simulink model "Router_communication"  (R2025a)
settings: Solver=VariableStepAuto  StartTime=0.0  StopTime=30  RelTol=1e-3
InitFcn:
  | %% Simulation parameters and waypoint trajectory
  | % Initial drone positions.
  | init_0=[0;0;0];
  | d_s=4;
  | init_1=init_0+d_s*[-1.1;0.1;0];
  | init_2=init_0+d_s*[0.3;-1.5;0];
  | init_3=init_0+d_s*[0.2;1.8;0];
  | init_4=init_0+d_s*[1.6;0.4;0];
  | 
  | Threshold = 1000*ones(45,1);
  | for i=1:9:37
  |     Threshold(i:i+2)=10;
  | end
  | gain_2=1;
  | 
  | % Router queues and background traffic.
  | router_buffer=5;
  | router_bandwith=20;
  | router_init_queue=3;
  | traffic_mean=20;
  | traffic_variance=1;
  | 
  | 
  | % Desired formation offsets.
  | init_f_0=[0;0;0];
  | d_f=1;
  | init_f_1=init_0+d_f*[-1;0;0];
  | init_f_2=init_0+d_f*[0;-1;0];
  | init_f_3=init_0+d_f*[0;1;0];
  | init_f_4=init_0+d_f*[1;0;0];
  | 
  | % Quadrotor mass and inertia.
  | mass = 1.2;
  | Ib   = diag([1.2416 1.2416 2*1.2416]);
  | 
  | % Time grid and waypoint trajectory.
  | Ts        = 0.001;
  | ttot      = 20;
  | tdead     = 10;
  | totalTime = ttot + tdead;
  | Nsamples  = 3000;
  | t_sample  = linspace(0, totalTime, Nsamples);
  | t=t_sample;
  | waypoints = [ ...
  |              0  0 -2 0;
  |              3  4 -5 0;
  |              2  1 -8 0;
  |              0 0 -10 0];
  | 
  | M    = size(waypoints,1);
  | t_wp = linspace(0, ttot, M);
  | 
  | p_d      = zeros(4, Nsamples);
  | dot_p_d  = zeros(4, Nsamples);
  | ddot_p_d = zeros(4, Nsamples);
  | 
  | idx_traj = t_sample <= ttot;
  | t_active = t_sample(idx_traj);
  | 
  | % Build position and yaw splines with zero endpoint velocities.
  | for dim = 1:4
  |     pp  = spline(t_wp, [0, waypoints(:,dim)&apos;, 0]);
  |     pp1 = fnder(pp,1);
  |     pp2 = fnder(pp,2);
  | 
  |     p_d(dim,    idx_traj) = ppval(pp,  t_active);
  |     dot_p_d(dim,idx_traj) = ppval(pp1, t_active);
  |     ddot_p_d(dim,idx_traj)= ppval(pp2, t_active);
  | end
  | 
  | % Hold the final waypoint after the maneuver.
  | last_wp_idx = M;
  | p_d(:, ~idx_traj)      = repmat(waypoints(last_wp_idx,:)&apos;, 1, sum(~idx_traj));
  | dot_p_d(:, ~idx_traj)  = 0;
  | ddot_p_d(:, ~idx_traj) = 0;
  | 
  | % Reference signals used by the Simulink blocks.
  | csi_d      = p_d(1:3,:);
  | psi_d      = p_d(4,:);
  | 
  | dot_csi_d  = dot_p_d(1:3,:);
  | ddot_csi_d = ddot_p_d(1:3,:);
  | dot_psi_d  = dot_p_d(4,:);
  | ddot_psi_d = ddot_p_d(4,:);
  | 
  | pos_0     = waypoints(1,1:3);
  | lin_vel_0 = [0 0 0];
  | w_bb_0    = [0 0 0];
undefined symbols (not defined in the file): A_diacenza, K
libraries: robotcorelib x5, dspsigops x1, uavutilslib x1
(part 1 of 3)
settings Model: Creator=fabioruggiero  LastModifiedBy=Giammo
settings ModelReferenceCC: EnableRefExpFcnMdlSchedulingChecks=on
settings RTWCC: GPUComputeCapability=3.5

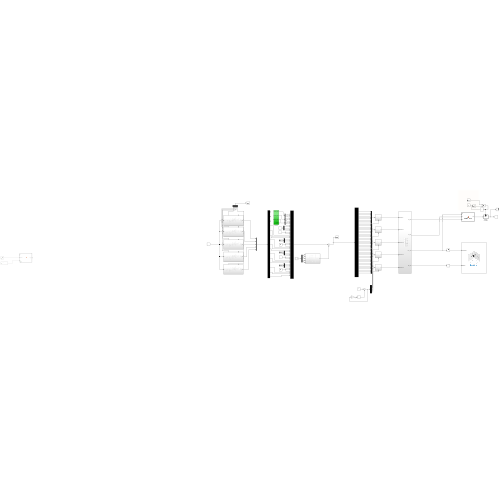
[thumbnail: Simulink's stored preview of the top-level diagram]
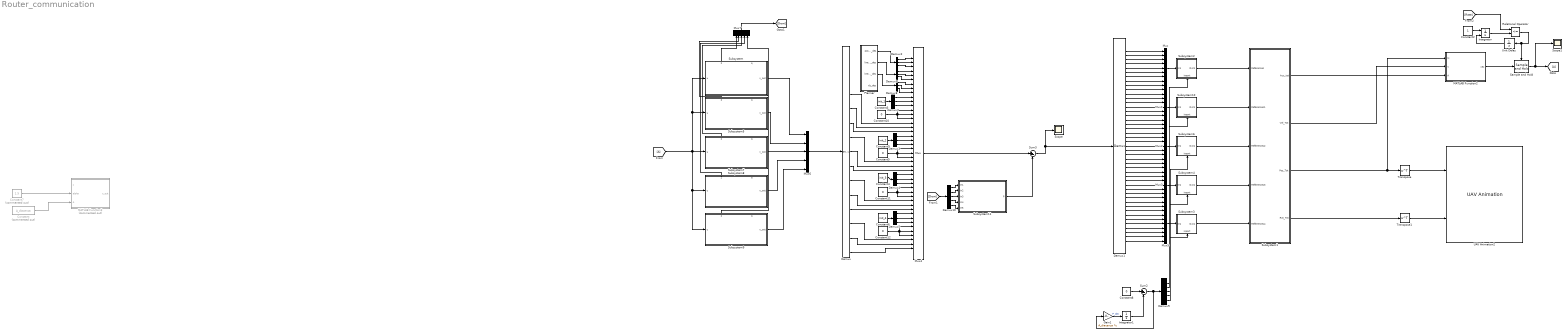
== system Router_communication ==
  Constant : Constant  Commented=on  Value=A_diacenza
  Constant{5,8,10..12} (5 alike) : Constant  Value=0
  Constant2 : Constant
  Constant3 : Constant  Value=init_1
  Constant4 : Constant  Value=init_3
  Constant6 : Constant  Value=init_4
  Constant7 : Constant  Commented=on  Value=1.5
  Constant9 : Constant  Value=init_2
  Demux : Demux  Outputs=15
  Demux1 : Demux  Outputs=45
  Demux10 : Demux  Outputs=5
  Demux{2..8} (7 alike) : Demux  Outputs=3
  Demux9 : Demux  Outputs=5
  From : From
  Gain1 : Gain  Gain=A_diacenza  Multiplication=Matrix(K*u)
  Goto : Goto
  Integrator : Integrator  ExternalReset=rising
  Integrator1 : Integrator
  MATLAB Function2 : MATLAB Function  TreatAsAtomicUnit=on
  MATLAB Function3 : MATLAB Function  Commented=on  TreatAsAtomicUnit=on
  Mux{,1..3,5} (5 alike) : Mux  Inputs=9
  Mux4 : Mux  Inputs=45
  Mux6 : Mux  Inputs=5
  Mux7 : Mux  Inputs=5
  Planner : Subsystem
  Relational Operator : RelationalOperator  Operator=<=  OutDataTypeStr=boolean  RndMeth=Simplest  InputSameDT=off
  Sample and Hold : dspsigops/Sample and Hold  trig=Rising edge  initCond=0  latchinput=off
  Scope : Scope
      settings: ActiveDisplayYMinimum=-34.636381337350009  ActiveDisplayYMaximum=35.165535436651609  DataLoggingVariableName=ScopeData6
  Scope1 : Scope
      settings: ActiveDisplayYMinimum=-11.627869915109368  ActiveDisplayYMaximum=11.845520962750264  DataLoggingVariableName=ScopeData33
  Subsystem : Subsystem
      settings: PortSchema="{\"entries\":[{\"content\":{\"sides\":[{\"content\":{\"connectorIds\":[\"In1\"]},\"type\":\"ConnectorPlacement.EquallySpacedRectSide\",\"uuid\":\"aabcef1b-4fc2-4bd0-92ff-98af5bae71df\"},{\"content\":{\"connectorIds\":[\"Out1\"],\"side\":\"RIGHT\"},\"type\":\"ConnectorPlacement.EquallySpacedRectSide\",\"uuid\":\"7f481425-bc3c-4684-b5b9-3c38277c27e3\"},{\"content\":{\"connectorIds\":[\"Out2\",\"Out3\"],\"side\":\"TOP\"},\"type\":\"ConnectorPlacement.EquallySpacedRectSide\",\"uuid\":\"89424cd8-205b-4e4e-84ff-a3a586731ce6\"}]},\"type\":\"ConnectorPlacement.EquallySpacedConnector\",\"uuid\":\"cde5d1e6-587e-462f-b172-cbaeaf24433c\"}],\"packageUris\":[\"http://schema.mathworks.com/mf0/Connector/R2020b\"],\"version\":\"1.0\"}"
  Subsystem1 : Subsystem
  Subsystem10 : Subsystem
      settings: PortSchema="{\"entries\":[{\"content\":{\"sides\":[{\"content\":{\"connectorIds\":[\"In1\"]},\"type\":\"ConnectorPlacement.EquallySpacedRectSide\",\"uuid\":\"6e5d8b99-8054-458f-abbe-7e3d6126420c\"},{\"content\":{\"connectorIds\":[\"Out1\"],\"side\":\"RIGHT\"},\"type\":\"ConnectorPlacement.EquallySpacedRectSide\",\"uuid\":\"d8af8c34-1227-4a19-bfdc-b42d943ed13c\"},{\"content\":{\"side\":\"TOP\"},\"type\":\"ConnectorPlacement.EquallySpacedRectSide\",\"uuid\":\"9c10b933-2873-4349-b535-f2af5c16ec70\"},{\"content\":{\"connectorIds\":[\"In2\"],\"side\":\"BOTTOM\"},\"type\":\"ConnectorPlacement.EquallySpacedRectSide\",\"uuid\":\"05be8d01-ed26-4f96-bcb1-0e501cb43bcc\"}]},\"type\":\"ConnectorPlacement.EquallySpacedConnector\",\"uuid\":\"f87e25de-488b-44c6-b2e5-9d22d609821c\"}],\"packageUris\":[\"http://schema.mathworks.com/mf0/Connector/R2020b\"],\"version\":\"1.0\"}"
  Subsystem11 : Subsystem
  Subsystem2 : Subsystem
      settings: PortSchema="{\"entries\":[{\"content\":{\"sides\":[{\"content\":{\"connectorIds\":[\"In1\"]},\"type\":\"ConnectorPlacement.EquallySpacedRectSide\",\"uuid\":\"6e5d8b99-8054-458f-abbe-7e3d6126420c\"},{\"content\":{\"connectorIds\":[\"Out1\"],\"side\":\"RIGHT\"},\"type\":\"ConnectorPlacement.EquallySpacedRectSide\",\"uuid\":\"d8af8c34-1227-4a19-bfdc-b42d943ed13c\"},{\"content\":{\"side\":\"TOP\"},\"type\":\"ConnectorPlacement.EquallySpacedRectSide\",\"uuid\":\"9c10b933-2873-4349-b535-f2af5c16ec70\"},{\"content\":{\"connectorIds\":[\"In2\"],\"side\":\"BOTTOM\"},\"type\":\"ConnectorPlacement.EquallySpacedRectSide\",\"uuid\":\"05be8d01-ed26-4f96-bcb1-0e501cb43bcc\"}]},\"type\":\"ConnectorPlacement.EquallySpacedConnector\",\"uuid\":\"f87e25de-488b-44c6-b2e5-9d22d609821c\"}],\"packageUris\":[\"http://schema.mathworks.com/mf0/Connector/R2020b\"],\"version\":\"1.0\"}"
  Subsystem3 : Subsystem
      settings: PortSchema="{\"entries\":[{\"content\":{\"sides\":[{\"content\":{\"connectorIds\":[\"In1\"]},\"type\":\"ConnectorPlacement.EquallySpacedRectSide\",\"uuid\":\"6e5d8b99-8054-458f-abbe-7e3d6126420c\"},{\"content\":{\"connectorIds\":[\"Out1\"],\"side\":\"RIGHT\"},\"type\":\"ConnectorPlacement.EquallySpacedRectSide\",\"uuid\":\"d8af8c34-1227-4a19-bfdc-b42d943ed13c\"},{\"content\":{\"side\":\"TOP\"},\"type\":\"ConnectorPlacement.EquallySpacedRectSide\",\"uuid\":\"9c10b933-2873-4349-b535-f2af5c16ec70\"},{\"content\":{\"connectorIds\":[\"In2\"],\"side\":\"BOTTOM\"},\"type\":\"ConnectorPlacement.EquallySpacedRectSide\",\"uuid\":\"05be8d01-ed26-4f96-bcb1-0e501cb43bcc\"}]},\"type\":\"ConnectorPlacement.EquallySpacedConnector\",\"uuid\":\"f87e25de-488b-44c6-b2e5-9d22d609821c\"}],\"packageUris\":[\"http://schema.mathworks.com/mf0/Connector/R2020b\"],\"version\":\"1.0\"}"
  Subsystem4 : Subsystem
      settings: PortSchema="{\"entries\":[{\"content\":{\"sides\":[{\"content\":{\"connectorIds\":[\"In1\"]},\"type\":\"ConnectorPlacement.EquallySpacedRectSide\",\"uuid\":\"6e5d8b99-8054-458f-abbe-7e3d6126420c\"},{\"content\":{\"connectorIds\":[\"Out1\"],\"side\":\"RIGHT\"},\"type\":\"ConnectorPlacement.EquallySpacedRectSide\",\"uuid\":\"d8af8c34-1227-4a19-bfdc-b42d943ed13c\"},{\"content\":{\"side\":\"TOP\"},\"type\":\"ConnectorPlacement.EquallySpacedRectSide\",\"uuid\":\"9c10b933-2873-4349-b535-f2af5c16ec70\"},{\"content\":{\"connectorIds\":[\"In2\"],\"side\":\"BOTTOM\"},\"type\":\"ConnectorPlacement.EquallySpacedRectSide\",\"uuid\":\"05be8d01-ed26-4f96-bcb1-0e501cb43bcc\"}]},\"type\":\"ConnectorPlacement.EquallySpacedConnector\",\"uuid\":\"f87e25de-488b-44c6-b2e5-9d22d609821c\"}],\"packageUris\":[\"http://schema.mathworks.com/mf0/Connector/R2020b\"],\"version\":\"1.0\"}"
  Subsystem5 : Subsystem
      settings: PortSchema="{\"entries\":[{\"content\":{\"sides\":[{\"content\":{\"connectorIds\":[\"In1\"]},\"type\":\"ConnectorPlacement.EquallySpacedRectSide\",\"uuid\":\"aabcef1b-4fc2-4bd0-92ff-98af5bae71df\"},{\"content\":{\"connectorIds\":[\"Out1\"],\"side\":\"RIGHT\"},\"type\":\"ConnectorPlacement.EquallySpacedRectSide\",\"uuid\":\"7f481425-bc3c-4684-b5b9-3c38277c27e3\"},{\"content\":{\"connectorIds\":[\"Out2\",\"Out3\"],\"side\":\"TOP\"},\"type\":\"ConnectorPlacement.EquallySpacedRectSide\",\"uuid\":\"89424cd8-205b-4e4e-84ff-a3a586731ce6\"}]},\"type\":\"ConnectorPlacement.EquallySpacedConnector\",\"uuid\":\"cde5d1e6-587e-462f-b172-cbaeaf24433c\"}],\"packageUris\":[\"http://schema.mathworks.com/mf0/Connector/R2020b\"],\"version\":\"1.0\"}"
  Subsystem6 : Subsystem
      settings: PortSchema="{\"entries\":[{\"content\":{\"sides\":[{\"content\":{\"connectorIds\":[\"In1\"]},\"type\":\"ConnectorPlacement.EquallySpacedRectSide\",\"uuid\":\"6e5d8b99-8054-458f-abbe-7e3d6126420c\"},{\"content\":{\"connectorIds\":[\"Out1\"],\"side\":\"RIGHT\"},\"type\":\"ConnectorPlacement.EquallySpacedRectSide\",\"uuid\":\"d8af8c34-1227-4a19-bfdc-b42d943ed13c\"},{\"content\":{\"side\":\"TOP\"},\"type\":\"ConnectorPlacement.EquallySpacedRectSide\",\"uuid\":\"9c10b933-2873-4349-b535-f2af5c16ec70\"},{\"content\":{\"connectorIds\":[\"In2\"],\"side\":\"BOTTOM\"},\"type\":\"ConnectorPlacement.EquallySpacedRectSide\",\"uuid\":\"05be8d01-ed26-4f96-bcb1-0e501cb43bcc\"}]},\"type\":\"ConnectorPlacement.EquallySpacedConnector\",\"uuid\":\"f87e25de-488b-44c6-b2e5-9d22d609821c\"}],\"packageUris\":[\"http://schema.mathworks.com/mf0/Connector/R2020b\"],\"version\":\"1.0\"}"
  Subsystem7 : Subsystem
      settings: PortSchema="{\"entries\":[{\"content\":{\"sides\":[{\"content\":{\"connectorIds\":[\"In1\"]},\"type\":\"ConnectorPlacement.EquallySpacedRectSide\",\"uuid\":\"aabcef1b-4fc2-4bd0-92ff-98af5bae71df\"},{\"content\":{\"connectorIds\":[\"Out1\"],\"side\":\"RIGHT\"},\"type\":\"ConnectorPlacement.EquallySpacedRectSide\",\"uuid\":\"7f481425-bc3c-4684-b5b9-3c38277c27e3\"},{\"content\":{\"connectorIds\":[\"Out2\",\"Out3\"],\"side\":\"TOP\"},\"type\":\"ConnectorPlacement.EquallySpacedRectSide\",\"uuid\":\"89424cd8-205b-4e4e-84ff-a3a586731ce6\"}]},\"type\":\"ConnectorPlacement.EquallySpacedConnector\",\"uuid\":\"cde5d1e6-587e-462f-b172-cbaeaf24433c\"}],\"packageUris\":[\"http://schema.mathworks.com/mf0/Connector/R2020b\"],\"version\":\"1.0\"}"
  Subsystem8 : Subsystem
      settings: PortSchema="{\"entries\":[{\"content\":{\"sides\":[{\"content\":{\"connectorIds\":[\"In1\"]},\"type\":\"ConnectorPlacement.EquallySpacedRectSide\",\"uuid\":\"aabcef1b-4fc2-4bd0-92ff-98af5bae71df\"},{\"content\":{\"connectorIds\":[\"Out1\"],\"side\":\"RIGHT\"},\"type\":\"ConnectorPlacement.EquallySpacedRectSide\",\"uuid\":\"7f481425-bc3c-4684-b5b9-3c38277c27e3\"},{\"content\":{\"connectorIds\":[\"Out2\",\"Out3\"],\"side\":\"TOP\"},\"type\":\"ConnectorPlacement.EquallySpacedRectSide\",\"uuid\":\"89424cd8-205b-4e4e-84ff-a3a586731ce6\"}]},\"type\":\"ConnectorPlacement.EquallySpacedConnector\",\"uuid\":\"cde5d1e6-587e-462f-b172-cbaeaf24433c\"}],\"packageUris\":[\"http://schema.mathworks.com/mf0/Connector/R2020b\"],\"version\":\"1.0\"}"
  Subsystem9 : Subsystem
      settings: PortSchema="{\"entries\":[{\"content\":{\"sides\":[{\"content\":{\"connectorIds\":[\"In1\"]},\"type\":\"ConnectorPlacement.EquallySpacedRectSide\",\"uuid\":\"c75a44b6-9c90-4115-8324-491a5ed9c89c\"},{\"content\":{\"connectorIds\":[\"Out1\"],\"side\":\"RIGHT\"},\"type\":\"ConnectorPlacement.EquallySpacedRectSide\",\"uuid\":\"690e00bc-d919-4544-9758-30244acb19c7\"},{\"content\":{\"connectorIds\":[\"Out2\",\"Out3\"],\"side\":\"TOP\"},\"type\":\"ConnectorPlacement.EquallySpacedRectSide\",\"uuid\":\"5c005ee2-f6aa-4388-a92a-4c7221a2c358\"}]},\"type\":\"ConnectorPlacement.EquallySpacedConnector\",\"uuid\":\"c7f8f7aa-2ed0-42e7-91ea-44ddde2a21e1\"}],\"packageUris\":[\"http://schema.mathworks.com/mf0/Connector/R2020b\"],\"version\":\"1.0\"}"
  Sum2 : Sum  Inputs=|+-
  Sum3 : Sum  Inputs=|+-
  Transpose : Math  Operator=transpose
  Transpose1 : Math  Operator=transpose
  UAV Animation2 : uavutilslib/UAV Animation  NumUAV=5  DynamicUAVConfig=off  UAVType=Multirotor  UAVSize=1  UAVColor=[1 0 0]  UAVTrajectoryAlpha=1  InertialZDirection=Down  RotationFormat=Quaternion  DrawMarkers=off  SampleTime=0.01
  Unit Delay : UnitDelay  SampleTime=Ts  HasFrameUpgradeWarning=on
  wires:
  Demux9/5 -> Subsystem3/2(Inport)
  Transpose1/1 -> UAV Animation2/2
  Transpose/1 -> UAV Animation2/1
  Sum2/1 -> Demux9/1, Gain1/1
  Gain1/1 -> Integrator1/1  "P_dot"
  Integrator1/1 -> Sum2/2
  Mux3/1 -> Subsystem4/1(In1)
  Mux/1 -> Subsystem2/1(In1)
  Subsystem2/1(Out1) -> Subsystem1/1(References)
  Demux9/2 -> Subsystem10/2(Inport)
  Subsystem3/1(Out1) -> Subsystem1/5(References4)
  Mux5/1 -> Subsystem3/1(In1)
  Subsystem6/1(Out1) -> Subsystem1/3(References2)
  Mux2/1 -> Subsystem6/1(In1)
  Demux1/1 -> Mux/1
  Demux1/15 -> Mux1/6
  Demux9/1 -> Subsystem2/2(Inport)
  Demux1/23 -> Mux2/5
  Demux1/12 -> Mux1/3
  Demux1/4 -> Mux/4
  Demux1/31 -> Mux3/4
  Demux1/41 -> Mux5/5
  Demux1/19 -> Mux2/1
  Demux1/26 -> Mux2/8
  Demux1/29 -> Mux3/2
  Demux1/34 -> Mux3/7
  Demux1/39 -> Mux5/3
  Demux1/20 -> Mux2/2
  Demux1/38 -> Mux5/2
  Demux1/43 -> Mux5/7
  Demux1/42 -> Mux5/6
  Demux1/30 -> Mux3/3
  Demux1/36 -> Mux3/9
  Demux1/27 -> Mux2/9
  Demux9/4 -> Subsystem4/2(Inport)
  Demux1/22 -> Mux2/4
  Demux1/32 -> Mux3/5
  Demux1/14 -> Mux1/5
  Demux1/13 -> Mux1/4
  Demux1/21 -> Mux2/3
  Demux1/33 -> Mux3/6
  Subsystem1/4(Rot_Tot) -> Transpose1/1
  Demux1/9 -> Mux/9
  Mux1/1 -> Subsystem10/1(In1)
  Demux1/40 -> Mux5/4
  Demux1/3 -> Mux/3
  Demux1/6 -> Mux/6
  Demux1/25 -> Mux2/7
  Demux1/8 -> Mux/8
  Demux1/28 -> Mux3/1
  Demux1/10 -> Mux1/1
  Demux1/7 -> Mux/7
  Demux1/37 -> Mux5/1
  Demux1/11 -> Mux1/2
  Demux1/45 -> Mux5/9
  Demux1/17 -> Mux1/8
  Demux1/35 -> Mux3/8
  Demux1/5 -> Mux/5
  Demux1/44 -> Mux5/8
  Constant11/1 -> Mux4/31, Mux4/33, Mux4/32
  Planner/3(linear_acceleration_des) -> Demux8/1
  Demux1/18 -> Mux1/9
  Demux/9 -> Mux4/27
  Demux1/16 -> Mux1/7
  Demux1/2 -> Mux/2
  Constant7/1 -> MATLAB Function3/2(alpha)
  Constant12/1 -> Mux4/40, Mux4/41, Mux4/42
  Constant10/1 -> Mux4/13, Mux4/15, Mux4/14
  Demux4/3 -> Mux4/30
  Mux4/1 -> Sum3/1
  Demux3/2 -> Mux4/20
  Demux2/2 -> Mux4/2
  Constant3/1 -> Demux7/1
  Demux5/2 -> Mux4/38
  Demux8/2 -> Mux4/8
  Constant8/1 -> Sum2/1
  Demux2/1 -> Mux4/1
  Demux7/2 -> Mux4/11
  Demux8/1 -> Mux4/7
  Demux2/3 -> Mux4/3
  Constant5/1 -> Mux4/22, Mux4/24, Mux4/23
  Demux/6 -> Mux4/18
  Demux3/3 -> Mux4/21
  Demux6/1 -> Mux4/4
  Demux/5 -> Mux4/17
  Demux8/3 -> Mux4/9
  Demux/12 -> Mux4/36
  Constant4/1 -> Demux4/1
  Demux6/2 -> Mux4/5
  Demux/7 -> Mux4/25
  Demux/14 -> Mux4/44
  Constant6/1 -> Demux5/1
  Constant9/1 -> Demux3/1
  Demux5/3 -> Mux4/39
  Demux/8 -> Mux4/26
  Demux7/1 -> Mux4/10
  Demux7/3 -> Mux4/12
  Planner/2(linear_velocity_des) -> Demux6/1
  Constant/1 -> MATLAB Function3/3(A)
  Sum3/1 -> Demux1/1, Scope/1
  Subsystem4/1(Out1) -> Subsystem1/4(References3)
  Demux3/1 -> Mux4/19
  Demux4/1 -> Mux4/28
  Demux4/2 -> Mux4/29
  Demux/10 -> Mux4/34
  Demux6/3 -> Mux4/6
  Demux/4 -> Mux4/16
  Planner/1(position_des) -> Demux2/1
  Demux5/1 -> Mux4/37
  Demux/11 -> Mux4/35
  Demux/15 -> Mux4/45
  Demux9/3 -> Subsystem6/2(Inport)
  Demux1/24 -> Mux2/6
  Subsystem10/1(Out1) -> Subsystem1/2(References1)
  Demux/13 -> Mux4/43
  Subsystem1/3(Pos_Tot) -> MATLAB Function2/1(M), Transpose/1
  Subsystem1/2(Vel_Tot) -> MATLAB Function2/2(V)
  Subsystem1/1(Acc_tot) -> MATLAB Function2/3(A)
  Mux6/1 -> Demux/1
  Subsystem/1(v_out) -> Mux6/1
  Subsystem5/1(v_out) -> Mux6/2
  Subsystem7/1(v_out) -> Mux6/3
  Subsystem8/1(v_out) -> Mux6/4
  Subsystem9/1(v_out) -> Mux6/5
  Subsystem11/1(P) -> Sum3/2
  Subsystem/2(" ") -> Mux7/1
  Demux10/1 -> Subsystem11/1(In1)
  Demux10/2 -> Subsystem11/2(In2)
  Demux10/3 -> Subsystem11/3(In3)
  Demux10/4 -> Subsystem11/4(In4)
  Demux10/5 -> Subsystem11/5(In5)
  Subsystem5/2(" ") -> Mux7/2
  Subsystem7/2(" ") -> Mux7/3
  Subsystem8/2(" ") -> Mux7/4
  Subsystem9/2(" ") -> Mux7/5
  Mux7/1 -> [Droni]
  [Droni] -> Demux10/1
  From/1 -> Subsystem7/1(u), Subsystem/1(u), Subsystem5/1(u), Subsystem8/1(u), Subsystem9/1(u)
  Constant2/1 -> Integrator/1
  Integrator/1 -> Relational Operator/2
  Relational Operator/1 -> Sample and Hold/Trigger, Unit Delay/1
  MATLAB Function2/1(vec) -> Sample and Hold/1
  Unit Delay/1 -> Integrator/2
  Sample and Hold/1 -> Scope1/1, Goto/1
  [Rate] -> Relational Operator/1

== system Router_communication/Planner ==
  Constant : Constant  Value=0
  Mux{1..4} (4 alike) : Mux  Inputs=3
  Trigonometric Function : Trigonometry
  Trigonometric Function1 : Trigonometry  Operator=cos
  ddot_x_d : FromWorkspace  VariableName=[t' ddot_csi_d(1,:)']  SampleTime=Ts
  ddot_y_d : FromWorkspace  VariableName=[t' ddot_csi_d(2,:)']  SampleTime=Ts
  ddot_z_d : FromWorkspace  VariableName=[t' ddot_csi_d(3,:)']  SampleTime=Ts
  dot_x_d1 : FromWorkspace  VariableName=[t' dot_csi_d(1,:)']  SampleTime=Ts
  dot_y_d1 : FromWorkspace  VariableName=[t' dot_csi_d(2,:)']  SampleTime=Ts
  dot_z_d1 : FromWorkspace  VariableName=[t' dot_csi_d(3,:)']  SampleTime=Ts
  psi_d1 : FromWorkspace  VariableName=[t' psi_d']  SampleTime=Ts
  x_d : FromWorkspace  VariableName=[t' csi_d(1,:)']  SampleTime=Ts
  y_d : FromWorkspace  VariableName=[t' csi_d(2,:)']  SampleTime=Ts
  z_d : FromWorkspace  VariableName=[t' csi_d(3,:)']  SampleTime=Ts
  position_des : Outport
  linear_velocity_des : Outport  Port=2
  linear_acceleration_des : Outport  Port=3
  xb_des : Outport  Port=4
  wires:
  y_d/1 -> Mux1/2
  z_d/1 -> Mux1/3
  x_d/1 -> Mux1/1
  ddot_y_d/1 -> Mux2/2
  ddot_z_d/1 -> Mux2/3
  ddot_x_d/1 -> Mux2/1
  Mux2/1 -> linear_acceleration_des/1
  Mux1/1 -> position_des/1
  dot_y_d1/1 -> Mux3/2
  dot_z_d1/1 -> Mux3/3
  dot_x_d1/1 -> Mux3/1
  Mux3/1 -> linear_velocity_des/1
  Mux4/1 -> xb_des/1
  Trigonometric Function/1 -> Mux4/2
  psi_d1/1 -> Trigonometric Function/1, Trigonometric Function1/1
  Trigonometric Function1/1 -> Mux4/1
  Constant/1 -> Mux4/3

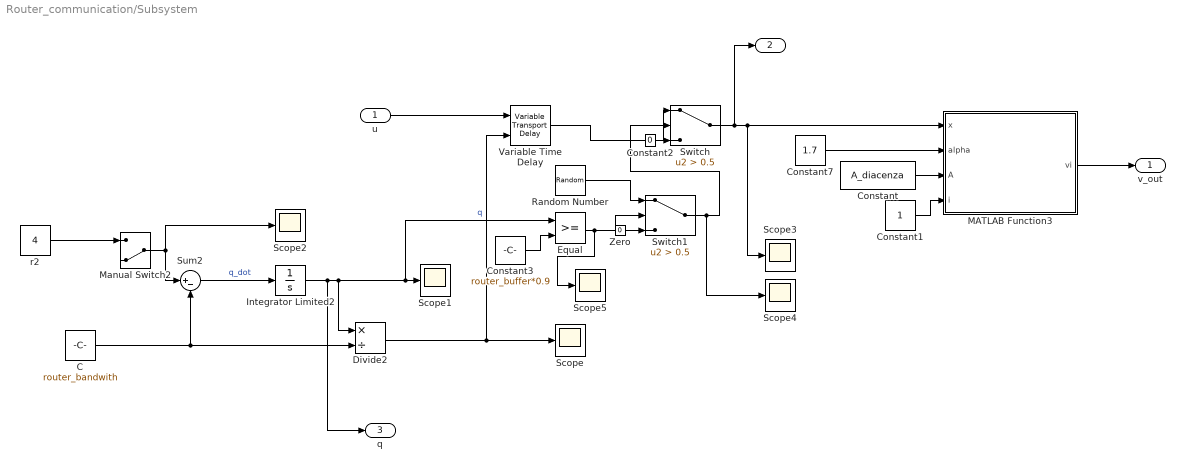
== system Router_communication/Subsystem ==
  u : Inport
  C : Constant  Value=router_bandwith
  Constant : Constant  Value=A_diacenza
  Constant1 : Constant
  Constant2 : Constant  Value=0
  Constant3 : Constant  Value=router_buffer*0.9
  Constant7 : Constant  Value=1.7
  Divide2 : Product  Inputs=*/
  Equal : RelationalOperator  OutDataTypeStr=boolean  RndMeth=Simplest  InputSameDT=off
  Integrator Limited2 : Integrator  InitialCondition=router_init_queue  LimitOutput=on  UpperSaturationLimit=router_buffer  LowerSaturationLimit=0
  MATLAB Function3 : MATLAB Function  TreatAsAtomicUnit=on
  Manual Switch2 : ManualSwitch  CurrentSetting=0
  Random Number : RandomNumber  Mean=0.5  SampleTime=0.1
  Scope{,1..5} (6 alike) : Scope
      Scope settings: ActiveDisplayYMinimum=0.1590289216839415  ActiveDisplayYMaximum=0.16563506037620399  DataLoggingVariableName=ScopeData7
      Scope1 settings: ActiveDisplayYMinimum=-1  ActiveDisplayYMaximum=1  DataLoggingVariableName=ScopeData8
      Scope2 settings: ActiveDisplayYMinimum=-4.9431007592698686  ActiveDisplayYMaximum=10.428917159954647  DataLoggingVariableName=ScopeData13
      Scope3 settings: ActiveDisplayYMinimum=-158.42328908870167  ActiveDisplayYMaximum=167.3995112416481  DataLoggingVariableName=ScopeData14
      Scope4 settings: ActiveDisplayYMinimum=-1  ActiveDisplayYMaximum=1  DataLoggingVariableName=ScopeData17
      Scope5 settings: ActiveDisplayYMinimum=-1  ActiveDisplayYMaximum=1  DataLoggingVariableName=ScopeData32
  Sum2 : Sum  Inputs=|+-
  Switch : Switch  Criteria=u2 > Threshold  Threshold=0.5  SaturateOnIntegerOverflow=off  InputSameDT=off
  Switch1 : Switch  Criteria=u2 > Threshold  Threshold=0.5  SaturateOnIntegerOverflow=off  InputSameDT=off
  Variable Time Delay : VariableTransportDelay  MaximumDelay=1000  InitialOutput=[init_0;zeros(6,1);init_1;zeros(6,1);init_2;zeros(6,1);init_3;zeros(6,1);init_4;zeros(6,1);]  MaximumPoints=1e4  ZeroDelay=on
  Zero : Constant  Value=0  OutDataTypeStr=Inherit: Inherit via back propagation
  r2 : Constant  Value=4
  v_out : Outport
  " " : Outport  Port=2
  q : Outport  Port=3
  wires:
  Constant7/1 -> MATLAB Function3/2(alpha)
  Constant/1 -> MATLAB Function3/3(A)
  Constant1/1 -> MATLAB Function3/4(i)
  MATLAB Function3/1(vi) -> v_out/1
  Constant3/1 -> Equal/2
  Zero/1 -> Switch1/3
  Integrator Limited2/1 -> q/1, Equal/1, Scope1/1, Divide2/1  "q"
  Switch/1 -> " "/1, MATLAB Function3/1(x), Scope3/1
  u/1 -> Variable Time Delay/1
  Sum2/1 -> Integrator Limited2/1  "q_dot"
  Divide2/1 -> Variable Time Delay/2, Scope/1
  r2/1 -> Manual Switch2/1
  Manual Switch2/1 -> Sum2/1, Scope2/1
  C/1 -> Divide2/2, Sum2/2
  Switch1/1 -> Scope4/1, Switch/2
  Variable Time Delay/1 -> Switch/3
  Constant2/1 -> Switch/1
  Random Number/1 -> Switch1/1
  Equal/1 -> Scope5/1, Switch1/2

== system Router_communication/Subsystem1 ==
  References : Inport
  References1 : Inport  Port=2
  References2 : Inport  Port=3
  References3 : Inport  Port=4
  References4 : Inport  Port=5
  Subsystem : Subsystem
  Subsystem1 : Subsystem
  Subsystem2 : Subsystem
  Subsystem3 : Subsystem
  Subsystem_1 : Subsystem
  Subsystem_2 : Subsystem
  Subsystem_3 : Subsystem
  Subsystem_4 : Subsystem
  Subsystem_5 : Subsystem
  Acc_tot : Outport
  Vel_Tot : Outport  Port=2
  Pos_Tot : Outport  Port=3
  Rot_Tot : Outport  Port=4
  wires:
  References1/1 -> Subsystem_2/1(References)
  References2/1 -> Subsystem_3/1(References)
  References3/1 -> Subsystem_4/1(References)
  References/1 -> Subsystem_1/1(References)
  References4/1 -> Subsystem_5/1(References)
  Subsystem_1/2(Lin Vel) -> Subsystem/1(In1)
  Subsystem_2/2(Lin Vel) -> Subsystem/2(In2)
  Subsystem_3/2(Lin Vel) -> Subsystem/3(In3)
  Subsystem_4/2(Lin Vel) -> Subsystem/4(In4)
  Subsystem_5/2(Lin Vel) -> Subsystem/5(In5)
  Subsystem/1(Out1) -> Vel_Tot/1
  Subsystem_1/3(Lin Pos) -> Subsystem1/1(In1)
  Subsystem_2/3(Lin Pos) -> Subsystem1/2(In2)
  Subsystem_3/3(Lin Pos) -> Subsystem1/3(In3)
  Subsystem_4/3(Lin Pos) -> Subsystem1/4(In4)
  Subsystem_5/3(Lin Pos) -> Subsystem1/5(In5)
  Subsystem1/1(Out1) -> Pos_Tot/1
  Subsystem_1/4(Rotation) -> Subsystem2/1(In1)
  Subsystem_2/4(Rotation) -> Subsystem2/2(In2)
  Subsystem_3/4(Rotation) -> Subsystem2/3(In3)
  Subsystem_4/4(Rotation) -> Subsystem2/4(In4)
  Subsystem_5/4(Rotation) -> Subsystem2/5(In5)
  Subsystem2/1(Out1) -> Rot_Tot/1
  Subsystem_1/1(Lin Acc) -> Subsystem3/1(In1)
  Subsystem_2/1(Lin Acc) -> Subsystem3/2(In2)
  Subsystem_3/1(Lin Acc) -> Subsystem3/3(In3)
  Subsystem_4/1(Lin Acc) -> Subsystem3/4(In4)
  Subsystem_5/1(Lin Acc) -> Subsystem3/5(In5)
  Subsystem3/1(Out1) -> Acc_tot/1

== system Router_communication/Subsystem10 ==
  In1 : Inport
  Inport : Inport  Port=2
  Constant1 : Constant  Value=[0;0;0]
  Demux : Demux  Outputs=9
  Demux1 : Demux  Outputs=3
  Mux : Mux  Inputs=3
  Mux2 : Mux  Inputs=10
  Sum : Sum  Inputs=++|
  Out1 : Outport
  wires:
  Mux2/1 -> Out1/1
  In1/1 -> Demux/1
  Demux/4 -> Mux2/4
  Demux/5 -> Mux2/5
  Demux/6 -> Mux2/6
  Demux/7 -> Mux2/7
  Demux/8 -> Mux2/8
  Demux/9 -> Mux2/9
  Demux/1 -> Mux/1
  Demux/2 -> Mux/2
  Demux/3 -> Mux/3
  Mux/1 -> Sum/2
  Constant1/1 -> Sum/1
  Sum/1 -> Demux1/1
  Demux1/1 -> Mux2/1
  Demux1/2 -> Mux2/2
  Demux1/3 -> Mux2/3
  Inport/1 -> Mux2/10

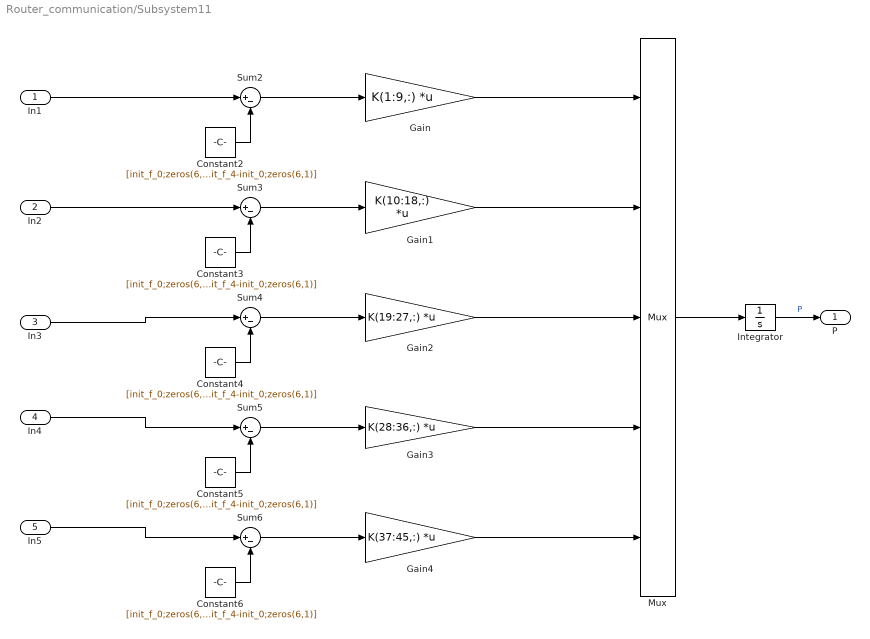
== system Router_communication/Subsystem11 ==
  In1 : Inport
  In2 : Inport  Port=2
  In3 : Inport  Port=3
  In4 : Inport  Port=4
  In5 : Inport  Port=5
  Constant{2..6} (5 alike) : Constant  Value=[init_f_0;zeros(6,1);init_f_1-init_0;zeros(6,1);init_f_2-init_0;zeros(6,1);init_f_3-init_0;zeros(6,1);init_f_4-init_0;zeros(6,1)]
  Gain : Gain  Gain=K(1:9,:)  Multiplication=Matrix(K*u)
  Gain1 : Gain  Gain=K(10:18,:)  Multiplication=Matrix(K*u)
  Gain2 : Gain  Gain=K(19:27,:)  Multiplication=Matrix(K*u)
  Gain3 : Gain  Gain=K(28:36,:)  Multiplication=Matrix(K*u)
  Gain4 : Gain  Gain=K(37:45,:)  Multiplication=Matrix(K*u)
  Integrator : Integrator
  Mux : Mux  Inputs=5
  Sum{2..6} (5 alike) : Sum  Inputs=|+-
  P : Outport
  wires:
  Integrator/1 -> P/1  "P"
  Constant2/1 -> Sum2/2
  Constant3/1 -> Sum3/2
  Constant4/1 -> Sum4/2
  Constant5/1 -> Sum5/2
  Constant6/1 -> Sum6/2
  Sum2/1 -> Gain/1
  Sum3/1 -> Gain1/1
  Sum4/1 -> Gain2/1
  Sum5/1 -> Gain3/1
  Sum6/1 -> Gain4/1
  Gain/1 -> Mux/1
  Gain1/1 -> Mux/2
  Gain2/1 -> Mux/3
  Gain3/1 -> Mux/4
  Gain4/1 -> Mux/5
  Mux/1 -> Integrator/1
  In1/1 -> Sum2/1
  In2/1 -> Sum3/1
  In3/1 -> Sum4/1
  In4/1 -> Sum5/1
  In5/1 -> Sum6/1

== system Router_communication/Subsystem2 ==
  In1 : Inport
  Inport : Inport  Port=2
  Constant1 : Constant  Value=[0;0;0]
  Demux : Demux  Outputs=9
  Demux1 : Demux  Outputs=3
  Mux : Mux  Inputs=3
  Mux2 : Mux  Inputs=10
  Sum : Sum  Inputs=++|
  Out1 : Outport
  wires:
  Mux2/1 -> Out1/1
  In1/1 -> Demux/1
  Demux/4 -> Mux2/4
  Demux/5 -> Mux2/5
  Demux/6 -> Mux2/6
  Demux/7 -> Mux2/7
  Demux/8 -> Mux2/8
  Demux/9 -> Mux2/9
  Demux/1 -> Mux/1
  Demux/2 -> Mux/2
  Demux/3 -> Mux/3
  Mux/1 -> Sum/2
  Constant1/1 -> Sum/1
  Sum/1 -> Demux1/1
  Demux1/1 -> Mux2/1
  Demux1/2 -> Mux2/2
  Demux1/3 -> Mux2/3
  Inport/1 -> Mux2/10

== system Router_communication/Subsystem3 ==
  In1 : Inport
  Inport : Inport  Port=2
  Constant1 : Constant  Value=[0;0;0]
  Demux : Demux  Outputs=9
  Demux1 : Demux  Outputs=3
  Mux : Mux  Inputs=3
  Mux2 : Mux  Inputs=10
  Sum : Sum  Inputs=++|
  Out1 : Outport
  wires:
  Mux2/1 -> Out1/1
  In1/1 -> Demux/1
  Demux/4 -> Mux2/4
  Demux/5 -> Mux2/5
  Demux/6 -> Mux2/6
  Demux/7 -> Mux2/7
  Demux/8 -> Mux2/8
  Demux/9 -> Mux2/9
  Demux/1 -> Mux/1
  Demux/2 -> Mux/2
  Demux/3 -> Mux/3
  Mux/1 -> Sum/2
  Constant1/1 -> Sum/1
  Sum/1 -> Demux1/1
  Demux1/1 -> Mux2/1
  Demux1/2 -> Mux2/2
  Demux1/3 -> Mux2/3
  Inport/1 -> Mux2/10

== system Router_communication/Subsystem4 ==
  In1 : Inport
  Inport : Inport  Port=2
  Constant1 : Constant  Value=[0;0;0]
  Demux : Demux  Outputs=9
  Demux1 : Demux  Outputs=3
  Mux : Mux  Inputs=3
  Mux2 : Mux  Inputs=10
  Sum : Sum  Inputs=++|
  Out1 : Outport
  wires:
  Mux2/1 -> Out1/1
  In1/1 -> Demux/1
  Demux/4 -> Mux2/4
  Demux/5 -> Mux2/5
  Demux/6 -> Mux2/6
  Demux/7 -> Mux2/7
  Demux/8 -> Mux2/8
  Demux/9 -> Mux2/9
  Demux/1 -> Mux/1
  Demux/2 -> Mux/2
  Demux/3 -> Mux/3
  Mux/1 -> Sum/2
  Constant1/1 -> Sum/1
  Sum/1 -> Demux1/1
  Demux1/1 -> Mux2/1
  Demux1/2 -> Mux2/2
  Demux1/3 -> Mux2/3
  Inport/1 -> Mux2/10

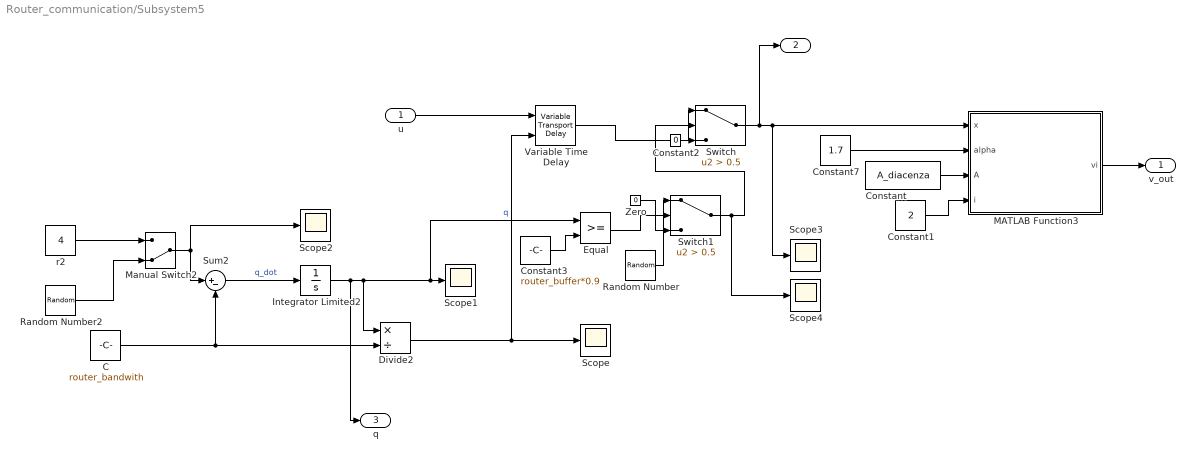
== system Router_communication/Subsystem5 ==
  u : Inport
  C : Constant  Value=router_bandwith
  Constant : Constant  Value=A_diacenza
  Constant1 : Constant  Value=2
  Constant2 : Constant  Value=0
  Constant3 : Constant  Value=router_buffer*0.9
  Constant7 : Constant  Value=1.7
  Divide2 : Product  Inputs=*/
  Equal : RelationalOperator  OutDataTypeStr=boolean  RndMeth=Simplest  InputSameDT=off
  Integrator Limited2 : Integrator  InitialCondition=router_init_queue  LimitOutput=on  UpperSaturationLimit=router_buffer  LowerSaturationLimit=0
  MATLAB Function3 : MATLAB Function  TreatAsAtomicUnit=on
  Manual Switch2 : ManualSwitch  CurrentSetting=0
  Random Number : RandomNumber  Mean=0.5  SampleTime=0.1
  Random Number2 : RandomNumber  Mean=traffic_mean  Variance=traffic_variance  Seed=21  SampleTime=Ts
  Scope{,1..4} (5 alike) : Scope
      Scope settings: ActiveDisplayYMinimum=-1  ActiveDisplayYMaximum=1  DataLoggingVariableName=ScopeData9
      Scope1 settings: ActiveDisplayYMinimum=-1  ActiveDisplayYMaximum=1  DataLoggingVariableName=ScopeData10
      Scope2 settings: ActiveDisplayYMinimum=-4.9431007592698686  ActiveDisplayYMaximum=10.428917159954647  DataLoggingVariableName=ScopeData18
      Scope3 settings: DataLoggingVariableName=ScopeData30
      Scope4 settings: DataLoggingVariableName=ScopeData31
  Sum2 : Sum  Inputs=|+-
  Switch : Switch  Criteria=u2 > Threshold  Threshold=0.5  SaturateOnIntegerOverflow=off  InputSameDT=off
  Switch1 : Switch  Criteria=u2 > Threshold  Threshold=0.5  SaturateOnIntegerOverflow=off  InputSameDT=off
  Variable Time Delay : VariableTransportDelay  MaximumDelay=1000  InitialOutput=[init_0;zeros(6,1);init_1;zeros(6,1);init_2;zeros(6,1);init_3;zeros(6,1);init_4;zeros(6,1);]  MaximumPoints=1e4  ZeroDelay=on
  Zero : Constant  Value=0  OutDataTypeStr=Inherit: Inherit via back propagation
  r2 : Constant  Value=4
  v_out : Outport
  " " : Outport  Port=2
  q : Outport  Port=3
  wires:
  Constant1/1 -> MATLAB Function3/4(i)
  Constant7/1 -> MATLAB Function3/2(alpha)
  Constant/1 -> MATLAB Function3/3(A)
  MATLAB Function3/1(vi) -> v_out/1
  Constant3/1 -> Equal/2
  Zero/1 -> Switch1/3
  Integrator Limited2/1 -> q/1, Equal/1, Scope1/1, Divide2/1  "q"
  Switch/1 -> " "/1, MATLAB Function3/1(x), Scope3/1
  u/1 -> Variable Time Delay/1
  Sum2/1 -> Integrator Limited2/1  "q_dot"
  Divide2/1 -> Variable Time Delay/2, Scope/1
  r2/1 -> Manual Switch2/1
  Random Number2/1 -> Manual Switch2/2
  Manual Switch2/1 -> Sum2/1, Scope2/1
  C/1 -> Divide2/2, Sum2/2
  Switch1/1 -> Scope4/1, Switch/2
  Variable Time Delay/1 -> Switch/3
  Equal/1 -> Switch1/2
  Constant2/1 -> Switch/1
  Random Number/1 -> Switch1/1

== system Router_communication/Subsystem6 ==
  In1 : Inport
  Inport : Inport  Port=2
  Constant1 : Constant  Value=[0;0;0]
  Demux : Demux  Outputs=9
  Demux1 : Demux  Outputs=3
  Mux : Mux  Inputs=3
  Mux2 : Mux  Inputs=10
  Sum : Sum  Inputs=++|
  Out1 : Outport
  wires:
  Mux2/1 -> Out1/1
  In1/1 -> Demux/1
  Demux/4 -> Mux2/4
  Demux/5 -> Mux2/5
  Demux/6 -> Mux2/6
  Demux/7 -> Mux2/7
  Demux/8 -> Mux2/8
  Demux/9 -> Mux2/9
  Demux/1 -> Mux/1
  Demux/2 -> Mux/2
  Demux/3 -> Mux/3
  Mux/1 -> Sum/2
  Constant1/1 -> Sum/1
  Sum/1 -> Demux1/1
  Demux1/1 -> Mux2/1
  Demux1/2 -> Mux2/2
  Demux1/3 -> Mux2/3
  Inport/1 -> Mux2/10

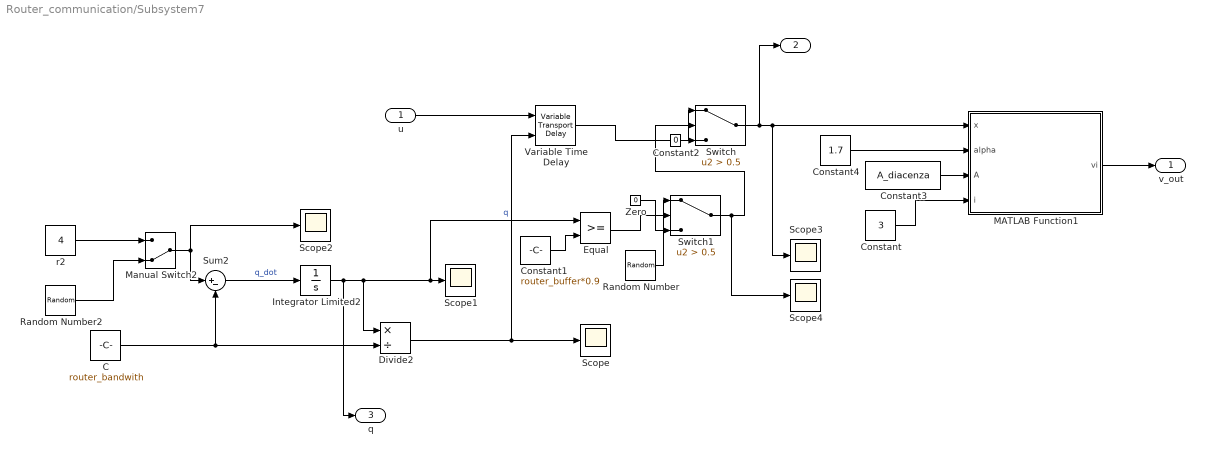
== system Router_communication/Subsystem7 ==
  u : Inport
  C : Constant  Value=router_bandwith
  Constant : Constant  Value=3
  Constant1 : Constant  Value=router_buffer*0.9
  Constant2 : Constant  Value=0
  Constant3 : Constant  Value=A_diacenza
  Constant4 : Constant  Value=1.7
  Divide2 : Product  Inputs=*/
  Equal : RelationalOperator  OutDataTypeStr=boolean  RndMeth=Simplest  InputSameDT=off
  Integrator Limited2 : Integrator  InitialCondition=router_init_queue  LimitOutput=on  UpperSaturationLimit=router_buffer  LowerSaturationLimit=0
  MATLAB Function1 : MATLAB Function  TreatAsAtomicUnit=on
  Manual Switch2 : ManualSwitch  CurrentSetting=0
  Random Number : RandomNumber  Mean=0.5  SampleTime=0.1
  Random Number2 : RandomNumber  Mean=traffic_mean  Variance=traffic_variance  Seed=21  SampleTime=Ts
  Scope{,1..4} (5 alike) : Scope
      Scope settings: ActiveDisplayYMinimum=-1  ActiveDisplayYMaximum=1  DataLoggingVariableName=ScopeData11
      Scope1 settings: ActiveDisplayYMinimum=-1  ActiveDisplayYMaximum=1  DataLoggingVariableName=ScopeData12
      Scope2 settings: ActiveDisplayYMinimum=-4.9431007592698686  ActiveDisplayYMaximum=10.428917159954647  DataLoggingVariableName=ScopeData19
      Scope3 settings: DataLoggingVariableName=ScopeData28
      Scope4 settings: DataLoggingVariableName=ScopeData29
  Sum2 : Sum  Inputs=|+-
  Switch : Switch  Criteria=u2 > Threshold  Threshold=0.5  SaturateOnIntegerOverflow=off  InputSameDT=off
  Switch1 : Switch  Criteria=u2 > Threshold  Threshold=0.5  SaturateOnIntegerOverflow=off  InputSameDT=off
  Variable Time Delay : VariableTransportDelay  MaximumDelay=1000  InitialOutput=[init_0;zeros(6,1);init_1;zeros(6,1);init_2;zeros(6,1);init_3;zeros(6,1);init_4;zeros(6,1);]  MaximumPoints=1e4  ZeroDelay=on
  Zero : Constant  Value=0  OutDataTypeStr=Inherit: Inherit via back propagation
  r2 : Constant  Value=4
  v_out : Outport
  " " : Outport  Port=2
  q : Outport  Port=3
  wires:
  Constant4/1 -> MATLAB Function1/2(alpha)
  MATLAB Function1/1(vi) -> v_out/1
  Constant3/1 -> MATLAB Function1/3(A)
  Constant/1 -> MATLAB Function1/4(i)
  Constant1/1 -> Equal/2
  Zero/1 -> Switch1/3
  Integrator Limited2/1 -> q/1, Equal/1, Scope1/1, Divide2/1  "q"
  Switch/1 -> " "/1, MATLAB Function1/1(x), Scope3/1
  u/1 -> Variable Time Delay/1
  Sum2/1 -> Integrator Limited2/1  "q_dot"
  Divide2/1 -> Variable Time Delay/2, Scope/1
  r2/1 -> Manual Switch2/1
  Random Number2/1 -> Manual Switch2/2
  Manual Switch2/1 -> Sum2/1, Scope2/1
  C/1 -> Divide2/2, Sum2/2
  Switch1/1 -> Scope4/1, Switch/2
  Variable Time Delay/1 -> Switch/3
  Equal/1 -> Switch1/2
  Constant2/1 -> Switch/1
  Random Number/1 -> Switch1/1

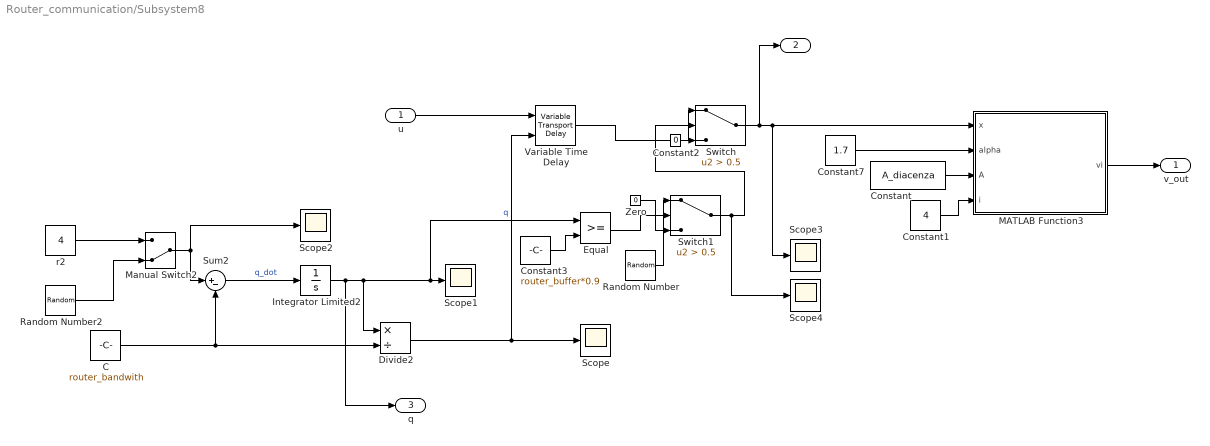
== system Router_communication/Subsystem8 ==
  u : Inport
  C : Constant  Value=router_bandwith
  Constant : Constant  Value=A_diacenza
  Constant1 : Constant  Value=4
  Constant2 : Constant  Value=0
  Constant3 : Constant  Value=router_buffer*0.9
  Constant7 : Constant  Value=1.7
  Divide2 : Product  Inputs=*/
  Equal : RelationalOperator  OutDataTypeStr=boolean  RndMeth=Simplest  InputSameDT=off
  Integrator Limited2 : Integrator  InitialCondition=router_init_queue  LimitOutput=on  UpperSaturationLimit=router_buffer  LowerSaturationLimit=0
  MATLAB Function3 : MATLAB Function  TreatAsAtomicUnit=on
  Manual Switch2 : ManualSwitch  CurrentSetting=0
  Random Number : RandomNumber  Mean=0.5  SampleTime=0.1
  Random Number2 : RandomNumber  Mean=traffic_mean  Variance=traffic_variance  Seed=21  SampleTime=Ts
  Scope{,1..4} (5 alike) : Scope
      Scope settings: ActiveDisplayYMinimum=-1  ActiveDisplayYMaximum=1  DataLoggingVariableName=ScopeData23
      Scope1 settings: ActiveDisplayYMinimum=-1  ActiveDisplayYMaximum=1  DataLoggingVariableName=ScopeData24
      Scope2 settings: ActiveDisplayYMinimum=-4.9431007592698686  ActiveDisplayYMaximum=10.428917159954647  DataLoggingVariableName=ScopeData25
      Scope3 settings: DataLoggingVariableName=ScopeData26
      Scope4 settings: DataLoggingVariableName=ScopeData27
  Sum2 : Sum  Inputs=|+-
  Switch : Switch  Criteria=u2 > Threshold  Threshold=0.5  SaturateOnIntegerOverflow=off  InputSameDT=off
  Switch1 : Switch  Criteria=u2 > Threshold  Threshold=0.5  SaturateOnIntegerOverflow=off  InputSameDT=off
  Variable Time Delay : VariableTransportDelay  MaximumDelay=1000  InitialOutput=[init_0;zeros(6,1);init_1;zeros(6,1);init_2;zeros(6,1);init_3;zeros(6,1);init_4;zeros(6,1);]  MaximumPoints=1e4  ZeroDelay=on
  Zero : Constant  Value=0  OutDataTypeStr=Inherit: Inherit via back propagation
  r2 : Constant  Value=4
  v_out : Outport
  " " : Outport  Port=2
  q : Outport  Port=3
  wires:
  Constant1/1 -> MATLAB Function3/4(i)
  Constant7/1 -> MATLAB Function3/2(alpha)
  MATLAB Function3/1(vi) -> v_out/1
  Constant/1 -> MATLAB Function3/3(A)
  Constant3/1 -> Equal/2
  Zero/1 -> Switch1/3
  Integrator Limited2/1 -> q/1, Equal/1, Scope1/1, Divide2/1  "q"
  Switch/1 -> " "/1, MATLAB Function3/1(x), Scope3/1
  u/1 -> Variable Time Delay/1
  Sum2/1 -> Integrator Limited2/1  "q_dot"
  Divide2/1 -> Variable Time Delay/2, Scope/1
  r2/1 -> Manual Switch2/1
  Random Number2/1 -> Manual Switch2/2
  Manual Switch2/1 -> Sum2/1, Scope2/1
  C/1 -> Divide2/2, Sum2/2
  Switch1/1 -> Scope4/1, Switch/2
  Variable Time Delay/1 -> Switch/3
  Equal/1 -> Switch1/2
  Constant2/1 -> Switch/1
  Random Number/1 -> Switch1/1

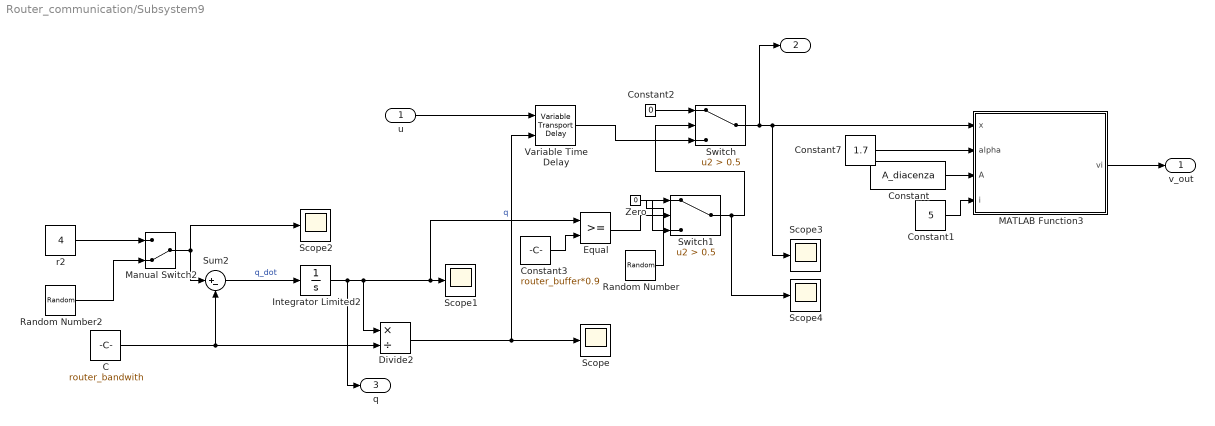
== system Router_communication/Subsystem9 ==
  u : Inport
  C : Constant  Value=router_bandwith
  Constant : Constant  Value=A_diacenza
  Constant1 : Constant  Value=5
  Constant2 : Constant  Value=0
  Constant3 : Constant  Value=router_buffer*0.9
  Constant7 : Constant  Value=1.7
  Divide2 : Product  Inputs=*/
  Equal : RelationalOperator  OutDataTypeStr=boolean  RndMeth=Simplest  InputSameDT=off
  Integrator Limited2 : Integrator  InitialCondition=router_init_queue  LimitOutput=on  UpperSaturationLimit=router_buffer  LowerSaturationLimit=0
  MATLAB Function3 : MATLAB Function  TreatAsAtomicUnit=on
  Manual Switch2 : ManualSwitch  CurrentSetting=0
  Random Number : RandomNumber  Mean=0.5  SampleTime=0.1
  Random Number2 : RandomNumber  Mean=traffic_mean  Variance=traffic_variance  Seed=21  SampleTime=Ts
  Scope{,1..4} (5 alike) : Scope
      Scope settings: ActiveDisplayYMinimum=-1  ActiveDisplayYMaximum=1  DataLoggingVariableName=ScopeData15
      Scope1 settings: ActiveDisplayYMinimum=-1  ActiveDisplayYMaximum=1  DataLoggingVariableName=ScopeData16
      Scope2 settings: ActiveDisplayYMinimum=-4.9431007592698686  ActiveDisplayYMaximum=10.428917159954647  DataLoggingVariableName=ScopeData21
      Scope3 settings: ActiveDisplayYMinimum=-1  ActiveDisplayYMaximum=1  DataLoggingVariableName=ScopeData20
      Scope4 settings: ActiveDisplayYMinimum=-1  ActiveDisplayYMaximum=1  DataLoggingVariableName=ScopeData22
  Sum2 : Sum  Inputs=|+-
  Switch : Switch  Criteria=u2 > Threshold  Threshold=0.5  SaturateOnIntegerOverflow=off  InputSameDT=off
  Switch1 : Switch  Criteria=u2 > Threshold  Threshold=0.5  SaturateOnIntegerOverflow=off  InputSameDT=off
  Variable Time Delay : VariableTransportDelay  MaximumDelay=1000  InitialOutput=[init_0;zeros(6,1);init_1;zeros(6,1);init_2;zeros(6,1);init_3;zeros(6,1);init_4;zeros(6,1);]  MaximumPoints=1e4  ZeroDelay=on
  Zero : Constant  Value=0  OutDataTypeStr=Inherit: Inherit via back propagation
  r2 : Constant  Value=4
  v_out : Outport
  " " : Outport  Port=2
  q : Outport  Port=3
  wires:
  u/1 -> Variable Time Delay/1
  Constant1/1 -> MATLAB Function3/4(i)
  C/1 -> Divide2/2, Sum2/2
  Divide2/1 -> Variable Time Delay/2, Scope/1
  Integrator Limited2/1 -> q/1, Equal/1, Scope1/1, Divide2/1  "q"
  Random Number2/1 -> Manual Switch2/2
  r2/1 -> Manual Switch2/1
  Sum2/1 -> Integrator Limited2/1  "q_dot"
  Manual Switch2/1 -> Sum2/1, Scope2/1
  Switch/1 -> " "/1, Scope3/1, MATLAB Function3/1(x)
  Constant7/1 -> MATLAB Function3/2(alpha)
  MATLAB Function3/1(vi) -> v_out/1
  Constant/1 -> MATLAB Function3/3(A)
  Variable Time Delay/1 -> Switch/3
  Constant2/1 -> Switch/1
  Constant3/1 -> Equal/2
  Equal/1 -> Switch1/2
  Zero/1 -> Switch1/3
  Switch1/1 -> Scope4/1, Switch/2
  Random Number/1 -> Switch1/1

== system Router_communication/Subsystem1/Subsystem ==
  In1 : Inport
  In2 : Inport  Port=2
  In3 : Inport  Port=3
  In4 : Inport  Port=4
  In5 : Inport  Port=5
  Matrix Concatenate2 : Concatenate  NumInputs=5  Mode=Multidimensional array  ConcatenateDimension=2
  Out1 : Outport
  wires:
  In3/1 -> Matrix Concatenate2/3
  In5/1 -> Matrix Concatenate2/5
  In4/1 -> Matrix Concatenate2/4
  In2/1 -> Matrix Concatenate2/2
  In1/1 -> Matrix Concatenate2/1
  Matrix Concatenate2/1 -> Out1/1

== system Router_communication/Subsystem1/Subsystem1 ==
  In1 : Inport
  In2 : Inport  Port=2
  In3 : Inport  Port=3
  In4 : Inport  Port=4
  In5 : Inport  Port=5
  Matrix Concatenate : Concatenate  NumInputs=5  Mode=Multidimensional array  ConcatenateDimension=2
  Out1 : Outport
  wires:
  In5/1 -> Matrix Concatenate/5
  Matrix Concatenate/1 -> Out1/1
  In2/1 -> Matrix Concatenate/2
  In3/1 -> Matrix Concatenate/3
  In1/1 -> Matrix Concatenate/1
  In4/1 -> Matrix Concatenate/4

== system Router_communication/Subsystem1/Subsystem2 ==
  In1 : Inport
  In2 : Inport  Port=2
  In3 : Inport  Port=3
  In4 : Inport  Port=4
  In5 : Inport  Port=5
  Matrix Concatenate1 : Concatenate  NumInputs=5  Mode=Multidimensional array  ConcatenateDimension=2
  Out1 : Outport
  wires:
  In4/1 -> Matrix Concatenate1/4
  In2/1 -> Matrix Concatenate1/2
  In5/1 -> Matrix Concatenate1/5
  Matrix Concatenate1/1 -> Out1/1
  In1/1 -> Matrix Concatenate1/1
  In3/1 -> Matrix Concatenate1/3

== system Router_communication/Subsystem1/Subsystem3 ==
  In1 : Inport
  In2 : Inport  Port=2
  In3 : Inport  Port=3
  In4 : Inport  Port=4
  In5 : Inport  Port=5
  Matrix Concatenate3 : Concatenate  NumInputs=5  Mode=Multidimensional array  ConcatenateDimension=2
  Out1 : Outport
  wires:
  In5/1 -> Matrix Concatenate3/5
  Matrix Concatenate3/1 -> Out1/1
  In3/1 -> Matrix Concatenate3/3
  In4/1 -> Matrix Concatenate3/4
  In2/1 -> Matrix Concatenate3/2
  In1/1 -> Matrix Concatenate3/1

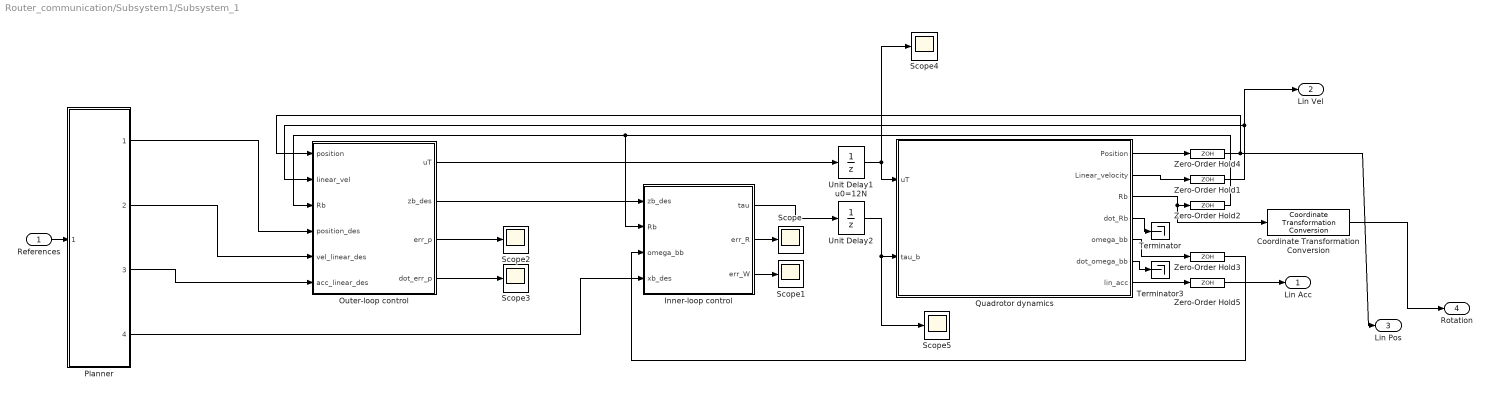
== system Router_communication/Subsystem1/Subsystem_1 ==
  References : Inport
  Coordinate Transformation Conversion : robotcorelib/Coordinate Transformation Conversion  InputRepresentation=Rotation Matrix  InputEulerSequence=ZYX  ShowTrVecInputPort=on  OutputRepresentation=Quaternion  OutputEulerSequence=ZYX  ShowTrVecOutputPort=on  SimulateUsing=Interpreted execution
  Inner-loop control : Subsystem
  Outer-loop control : MATLAB Function  TreatAsAtomicUnit=on
  Planner : Subsystem
  Quadrotor dynamics : Subsystem
  Scope{,1..5} (6 alike) : Scope
      Scope settings: ActiveDisplayYMinimum=-1.2E-5  ActiveDisplayYMaximum=1.2E-5
      Scope1 settings: ActiveDisplayYMinimum=-1.2E-5  ActiveDisplayYMaximum=1.2E-5
      Scope2 settings: ActiveDisplayYMinimum=-3.9E-5  ActiveDisplayYMaximum=1.1E-5  DataLoggingVariableName=ScopeData2
      Scope3 settings: ActiveDisplayYMinimum=-0.00022  ActiveDisplayYMaximum=0.00011  DataLoggingVariableName=ScopeData3
      Scope4 settings: ActiveDisplayYMinimum=11.66748  ActiveDisplayYMaximum=12.03695  DataLoggingVariableName=ScopeData4
      Scope5 settings: ActiveDisplayYMinimum=-0.02035  ActiveDisplayYMaximum=0.02036  DataLoggingVariableName=ScopeData5
  Terminator : Terminator
  Terminator3 : Terminator
  Unit Delay1 u0=12N : UnitDelay  InitialCondition=12  SampleTime=Ts
  Unit Delay2 : UnitDelay  InitialCondition=[0 0 0]  SampleTime=Ts
  Zero-Order Hold{1..5} (5 alike) : ZeroOrderHold  SampleTime=Ts
  Lin Acc : Outport
  Lin Vel : Outport  Port=2
  Lin Pos : Outport  Port=3
  Rotation : Outport  Port=4
  wires:
  Zero-Order Hold5/1 -> Lin Acc/1
  Quadrotor dynamics/7(lin_acc) -> Zero-Order Hold5/1
  Planner/1(position_des) -> Outer-loop control/4(position_des)
  Quadrotor dynamics/1(Position) -> Zero-Order Hold4/1
  Quadrotor dynamics/3(Rb) -> Zero-Order Hold2/1, Coordinate Transformation Conversion/1
  Quadrotor dynamics/4(dot_Rb) -> Terminator/1
  Planner/4(xb_des) -> Inner-loop control/4(xb_des)
  Inner-loop control/1(tau) -> Unit Delay2/1
  Planner/2(linear_velocity_des) -> Outer-loop control/5(vel_linear_des)
  Quadrotor dynamics/2(Linear_velocity) -> Zero-Order Hold1/1
  Quadrotor dynamics/6(dot_omega_bb) -> Terminator3/1
  Outer-loop control/3(err_p) -> Scope2/1
  Coordinate Transformation Conversion/1 -> Rotation/1
  Quadrotor dynamics/5(omega_bb) -> Zero-Order Hold3/1
  Zero-Order Hold2/1 -> Inner-loop control/2(Rb), Outer-loop control/3(Rb)
  References/1 -> Planner/1(References)
  Planner/3(linear_acceleration_des) -> Outer-loop control/6(acc_linear_des)
  Inner-loop control/3(err_W) -> Scope1/1
  Outer-loop control/2(zb_des) -> Inner-loop control/1(zb_des)
  Inner-loop control/2(err_R) -> Scope/1
  Outer-loop control/1(uT) -> Unit Delay1 u0=12N/1
  Unit Delay2/1 -> Quadrotor dynamics/2(tau_b), Scope5/1
  Zero-Order Hold3/1 -> Inner-loop control/3(omega_bb)
  Unit Delay1 u0=12N/1 -> Scope4/1, Quadrotor dynamics/1(uT)
  Outer-loop control/4(dot_err_p) -> Scope3/1
  Zero-Order Hold1/1 -> Outer-loop control/2(linear_vel), Lin Vel/1
  Zero-Order Hold4/1 -> Outer-loop control/1(position), Lin Pos/1

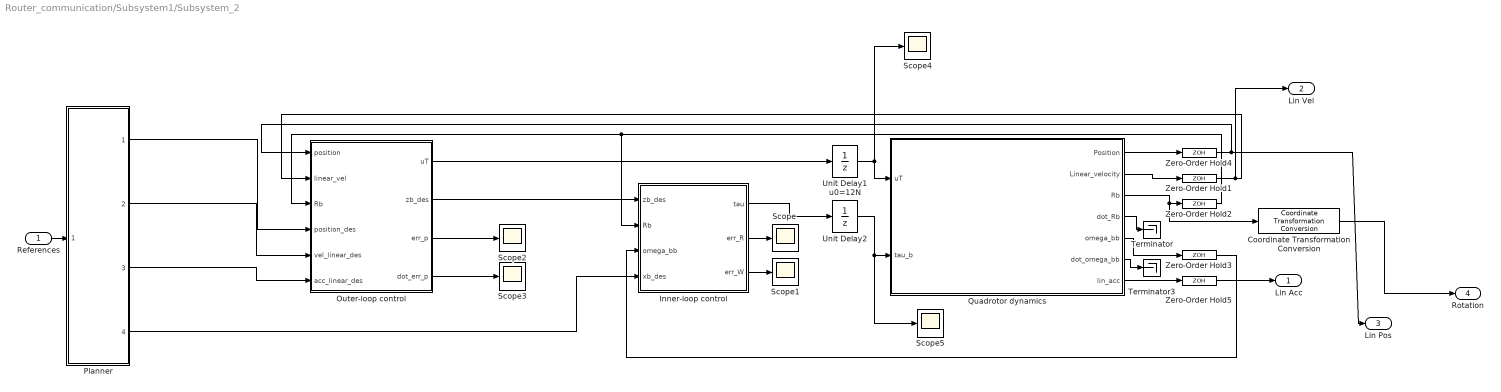
== system Router_communication/Subsystem1/Subsystem_2 ==
  References : Inport
  Coordinate Transformation Conversion : robotcorelib/Coordinate Transformation Conversion  InputRepresentation=Rotation Matrix  InputEulerSequence=ZYX  ShowTrVecInputPort=on  OutputRepresentation=Quaternion  OutputEulerSequence=ZYX  ShowTrVecOutputPort=on  SimulateUsing=Interpreted execution
  Inner-loop control : Subsystem
  Outer-loop control : MATLAB Function  TreatAsAtomicUnit=on
  Planner : Subsystem
  Quadrotor dynamics : Subsystem
  Scope{,1..5} (6 alike) : Scope
      Scope settings: ActiveDisplayYMinimum=-1.2E-5  ActiveDisplayYMaximum=1.2E-5
      Scope1 settings: ActiveDisplayYMinimum=-1.2E-5  ActiveDisplayYMaximum=1.2E-5
      Scope2 settings: ActiveDisplayYMinimum=-3.9E-5  ActiveDisplayYMaximum=1.1E-5  DataLoggingVariableName=ScopeData2
      Scope3 settings: ActiveDisplayYMinimum=-0.00022  ActiveDisplayYMaximum=0.00011  DataLoggingVariableName=ScopeData3
      Scope4 settings: ActiveDisplayYMinimum=11.66748  ActiveDisplayYMaximum=12.03695  DataLoggingVariableName=ScopeData4
      Scope5 settings: ActiveDisplayYMinimum=-0.02035  ActiveDisplayYMaximum=0.02036  DataLoggingVariableName=ScopeData5
  Terminator : Terminator
  Terminator3 : Terminator
  Unit Delay1 u0=12N : UnitDelay  InitialCondition=12  SampleTime=Ts
  Unit Delay2 : UnitDelay  InitialCondition=[0 0 0]  SampleTime=Ts
  Zero-Order Hold{1..5} (5 alike) : ZeroOrderHold  SampleTime=Ts
  Lin Acc : Outport
  Lin Vel : Outport  Port=2
  Lin Pos : Outport  Port=3
  Rotation : Outport  Port=4
  wires:
  Zero-Order Hold5/1 -> Lin Acc/1
  Quadrotor dynamics/7(lin_acc) -> Zero-Order Hold5/1
  Planner/1(position_des) -> Outer-loop control/4(position_des)
  Quadrotor dynamics/1(Position) -> Zero-Order Hold4/1
  Quadrotor dynamics/3(Rb) -> Zero-Order Hold2/1, Coordinate Transformation Conversion/1
  Quadrotor dynamics/4(dot_Rb) -> Terminator/1
  Planner/4(xb_des) -> Inner-loop control/4(xb_des)
  Inner-loop control/1(tau) -> Unit Delay2/1
  Planner/2(linear_velocity_des) -> Outer-loop control/5(vel_linear_des)
  Quadrotor dynamics/2(Linear_velocity) -> Zero-Order Hold1/1
  Quadrotor dynamics/6(dot_omega_bb) -> Terminator3/1
  Outer-loop control/3(err_p) -> Scope2/1
  Coordinate Transformation Conversion/1 -> Rotation/1
  Quadrotor dynamics/5(omega_bb) -> Zero-Order Hold3/1
  Zero-Order Hold2/1 -> Inner-loop control/2(Rb), Outer-loop control/3(Rb)
  References/1 -> Planner/1(References)
  Planner/3(linear_acceleration_des) -> Outer-loop control/6(acc_linear_des)
  Inner-loop control/3(err_W) -> Scope1/1
  Outer-loop control/2(zb_des) -> Inner-loop control/1(zb_des)
  Inner-loop control/2(err_R) -> Scope/1
  Outer-loop control/1(uT) -> Unit Delay1 u0=12N/1
  Unit Delay2/1 -> Quadrotor dynamics/2(tau_b), Scope5/1
  Zero-Order Hold3/1 -> Inner-loop control/3(omega_bb)
  Unit Delay1 u0=12N/1 -> Scope4/1, Quadrotor dynamics/1(uT)
  Outer-loop control/4(dot_err_p) -> Scope3/1
  Zero-Order Hold1/1 -> Outer-loop control/2(linear_vel), Lin Vel/1
  Zero-Order Hold4/1 -> Outer-loop control/1(position), Lin Pos/1
